simulink model "LQRconlacnguoc"  (R2024b)
settings: Solver=ode45  StartTime=0.0  StopTime=60  FixedStep=0.001  MaxStep=0.01  RelTol=1e-3
values from neighbouring files (symbols this model uses):
  D = [0; 0]    [K_vector_2.m]
libraries: simulink x20, slpidlib x11, slctrl_smc x5, mpclib x1, dspstat3 x1, rllib x1
(part 3 of 3)

== matlab function LQRconlacnguoc/Manual SMC Adaptive/Subsystem/MATLAB Function ==
  settings: updateMethod=DISCRETE  sampleTime=0.01
  data: s input; eta output; x input; x_ref input; phi output; C output
function [eta, phi, C] = culture_bees_smc(s, x, x_ref)

%% ── PREALLOCATE OUTPUTS ──────────────────────────────────────────────
eta = double(0);
phi = double(0);
C   = zeros(4, 1);

%% ── PERSISTENT STATE ─────────────────────────────────────────────────
persistent belief_lambda belief_alpha belief_mu
persistent norm_lambda norm_alpha norm_mu
persistent initialized

%% ── INITIALIZATION ───────────────────────────────────────────────────
if isempty(initialized)
    initialized   = int8(1);
    belief_lambda = double(8.0);
    belief_alpha  = double(20.0);
    belief_mu     = double(36.5);
    norm_lambda   = double([1.0,  15.0]);
    norm_alpha    = double([5.0,  25.0]);
    norm_mu       = double([10.0, 50.0]);
end

%% ── EXTRACT SCALARS ──────────────────────────────────────────────────
x2   = x(3);
xd2  = x(4);
x2r  = x_ref(3);
xd2r = x_ref(4);

e_pos = (x2r - x2)^2;
e_vel = (xd2r - xd2)^2;
e_tot = e_pos + e_vel;

%% ── DYNAMIC HARD FLOORS (key fix) ───────────────────────────────────
% Alpha floor scales directly with error magnitude
% When error is large, alpha CANNOT go below a meaningful minimum
% This replaces the soft adequacy penalty with a hard constraint
alpha_floor  = double(5.0) + double(15.0) * tanh(e_tot * 10.0);
% alpha_floor ≈ 5   when e_tot ≈ 0    (settled, allow alpha to relax)
% alpha_floor ≈ 20  when e_tot = 0.1  (moderate error, hold alpha high)
% alpha_floor ≈ 20  when e_tot large  (large error, maximum floor)

lambda_floor = double(1.0) + double(7.0)  * tanh(e_tot * 10.0);
% lambda_floor ≈ 1  when settled
% lambda_floor ≈ 8  when error present

% Enforce floors on belief state BEFORE optimization runs
% This prevents the optimizer from ever exploring below safe values
if belief_alpha < alpha_floor
    belief_alpha = alpha_floor;
end
if belief_lambda < lambda_floor
    belief_lambda = lambda_floor;
end

% Also enforce on normative bounds lower limit
current_alpha_min  = alpha_floor;
current_lambda_min = lambda_floor;

%% ── LOSS OF CONTROL RESET ────────────────────────────────────────────
control_lost = (e_tot > 0.005) && (belief_alpha < alpha_floor * 1.2);
if control_lost
    belief_lambda = double(8.0);
    belief_alpha  = double(20.0);
    belief_mu     = double(36.5);
    norm_lambda   = double([current_lambda_min, 15.0]);
    norm_alpha    = double([current_alpha_min,  25.0]);
    norm_mu       = double([10.0, 50.0]);
end

%% ── ALGORITHM HYPERPARAMETERS ────────────────────────────────────────
n_scout    = int32(10);
n_selected = int32(4);
n_recruit  = int32(20);
N_belief   = int32(5);

lambda_min = current_lambda_min;  lambda_max = double(15.0);
alpha_min  = current_alpha_min;   alpha_max  = double(25.0);
mu_min     = double(10.0);        mu_max     = double(50.0);

patch_alpha  = double(0.0125);
patch_lambda = double(0.0135);
patch_mu     = double(0.0175);

patch_c_alpha  = double(0.01);
patch_c_lambda = double(0.01);
patch_c_mu     = double(0.01);

%% ── PART 1: BREEDING ENGINE ──────────────────────────────────────────
scouts = zeros(n_scout, 3);
for i = 1:n_scout
    scouts(i,1) = norm_lambda(1) + rand()*(norm_lambda(2)-norm_lambda(1));
    scouts(i,2) = norm_alpha(1)  + rand()*(norm_alpha(2) -norm_alpha(1));
    scouts(i,3) = norm_mu(1)     + rand()*(norm_mu(2)    -norm_mu(1));
end

%% ── PART 2: SEARCH ENGINE ────────────────────────────────────────────
scout_mse = zeros(n_scout, 1);
for i = 1:n_scout
    scout_mse(i) = eval_mse(scouts(i,1), scouts(i,2), scouts(i,3), ...
                             s, x2, xd2, x2r, xd2r, e_tot, alpha_floor);
end

[~, idx]  = sort(scout_mse, 'ascend');
selected  = scouts(idx(1:n_selected), :);

best_recruit     = zeros(n_selected, 3);
best_recruit_mse = zeros(n_selected, 1);

for i = 1:n_selected
    site        = selected(i,:);
    recruits    = zeros(n_recruit, 3);
    recruit_mse = zeros(n_recruit, 1);

    for j = 1:n_recruit
        d_lambda = patch_lambda * site(1) * (rand() - 0.5);
        d_alpha  = patch_alpha  * site(2) * (rand() - 0.5);
        d_mu     = patch_mu     * site(3) * (rand() - 0.5);

        cl = clamp_val(site(1)+d_lambda, lambda_min, lambda_max);
        ca = clamp_val(site(2)+d_alpha,  alpha_min,  alpha_max);
        cm = clamp_val(site(3)+d_mu,     mu_min,     mu_max);

        recruits(j,:)  = [cl, ca, cm];
        recruit_mse(j) = eval_mse(cl, ca, cm, s, x2, xd2, x2r, xd2r, ...
                                   e_tot, alpha_floor);
    end

    [best_recruit_mse(i), best_j] = min(recruit_mse);
    best_recruit(i,:) = recruits(best_j,:);
end

[~, fittest_idx] = sort(best_recruit_mse, 'ascend');
fittest_bees     = best_recruit(fittest_idx, :);
fittest_mse_vec  = best_recruit_mse(fittest_idx);

%% ── PART 3: AGGREGATION KNOWLEDGE ENGINE ────────────────────────────
n_sc          = max(int32(1), round(0.4 * double(n_selected)));
scout_culture = fittest_bees(1:n_sc, :);
sc_mse        = fittest_mse_vec(1:n_sc);

n_scc       = max(int32(1), round(0.5 * double(n_sc)));
[~, sc_idx] = sort(sc_mse, 'ascend');
sel_culture = scout_culture(sc_idx(1:n_scc), :);

current_belief_mse = eval_mse(belief_lambda, belief_alpha, belief_mu, ...
                               s, x2, xd2, x2r, xd2r, e_tot, alpha_floor);
best_sc_mse = sc_mse(sc_idx(1));

if best_sc_mse < current_belief_mse
    belief_lambda = sel_culture(1,1);
    belief_alpha  = sel_culture(1,2);
    belief_mu     = sel_culture(1,3);
end

best_bl  = belief_lambda;
best_ba  = belief_alpha;
best_bm  = belief_mu;
best_mse = current_belief_mse;

for iter = 1:N_belief
    d_lc = patch_c_lambda * belief_lambda * (rand() - 0.5);
    d_ac = patch_c_alpha  * belief_alpha  * (rand() - 0.5);
    d_mc = patch_c_mu     * belief_mu     * (rand() - 0.5);

    cand_l = clamp_val(belief_lambda+d_lc, lambda_min, lambda_max);
    cand_a = clamp_val(belief_alpha +d_ac, alpha_min,  alpha_max);
    cand_m = clamp_val(belief_mu    +d_mc, mu_min,     mu_max);

    cand_mse = eval_mse(cand_l, cand_a, cand_m, s, x2, xd2, x2r, xd2r, ...
                         e_tot, alpha_floor);

    in_norm = (cand_l >= norm_lambda(1)) && (cand_l <= norm_lambda(2)) && ...
              (cand_a >= norm_alpha(1))  && (cand_a <= norm_alpha(2))  && ...
              (cand_m >= norm_mu(1))     && (cand_m <= norm_mu(2));

    if cand_mse < best_mse && in_norm
        best_bl  = cand_l;
        best_ba  = cand_a;
        best_bm  = cand_m;
        best_mse = cand_mse;
    end
end

% Update normative lower bounds to never go below current floors
norm_lambda = update_norm(norm_lambda, best_bl, lambda_min, lambda_max);
norm_alpha  = update_norm(norm_alpha,  best_ba, alpha_min,  alpha_max);
norm_mu     = update_norm(norm_mu,     best_bm, mu_min,     mu_max);

% Hard-enforce floors on updated bounds
if norm_lambda(1) < current_lambda_min
    norm_lambda(1) = current_lambda_min;
end
if norm_alpha(1) < current_alpha_min
    norm_alpha(1) = current_alpha_min;
end

belief_lambda = best_bl;
belief_alpha  = best_ba;
belief_mu     = best_bm;

%% ── FINAL FLOOR ENFORCEMENT ON OUTPUTS ──────────────────────────────
% Last line of defense — outputs never go below error-scaled floors
if belief_alpha  < alpha_floor;  belief_alpha  = alpha_floor;  end
if belief_lambda < lambda_floor; belief_lambda = lambda_floor; end

%% ── OUTPUT ASSIGNMENT ────────────────────────────────────────────────
eta = double(belief_alpha);
phi = double(1.0 / belief_mu);
C   = double(belief_lambda) .* [0.0; 1.0; 0.0; 1.0];

end

%% ════════════════════════════════════════════════════════════════════
%% LOCAL: MSE COST
%% ════════════════════════════════════════════════════════════════════
function mse = eval_mse(lambda, alpha, mu, s, x2, xd2, x2r, xd2r, ...
                         e_tot, alpha_floor)

    e_pos = (x2r - x2)^2;
    e_vel = (xd2r - xd2)^2;

    %% Term 1 — Tracking (primary)
    tracking = e_pos + e_vel;

    %% Term 2 — Surface penalty
    s_penalty = s^2;

    %% Term 3 — Alpha floor violation penalty
    % Heavily penalize any alpha below the error-scaled floor
    % This is what forces the optimizer to keep alpha adequate
    floor_violation = max(0.0, alpha_floor - alpha)^2 * 100.0;

    %% Term 4 — Chattering: only penalize when truly settled
    % settled = near surface AND near zero error simultaneously
    settled      = exp(-5.0 * abs(s)) * exp(-50.0 * e_tot);
    chat_penalty = alpha^2 * mu * settled * 0.0001;

    %% Term 5 — Lambda alignment with surface
    s_expected    = lambda * sqrt(e_pos + 0.0001) + sqrt(e_vel + 0.0001);
    align_penalty = (abs(s) - s_expected)^2 / (s_expected^2 + 0.01);

    %% Term 6 — Mu sizing (keep phi ≈ 0.0274, mu ≈ 36.5)
    % Penalize deviation from target mu
    mu_target   = double(36.5);
    mu_penalty  = (mu - mu_target)^2 / (mu_target^2) * 0.1;

    %% Weighted sum
    mse = 2.0  * tracking       ...
        + 0.3  * s_penalty      ...
        + 1.0  * floor_violation ...  % hardest constraint
        + 0.05 * chat_penalty   ...
        + 0.2  * align_penalty  ...
        + 0.1  * mu_penalty;

end

%% ════════════════════════════════════════════════════════════════════
%% LOCAL: CLAMP
%% ════════════════════════════════════════════════════════════════════
function val = clamp_val(val, lo, hi)
    if val < lo; val = lo; end
    if val > hi; val = hi; end
end

%% ════════════════════════════════════════════════════════════════════
%% LOCAL: NORMATIVE BOUNDS UPDATER
%% ════════════════════════════════════════════════════════════════════
function bounds = update_norm(bounds, best_val, hard_min, hard_max)
    shrink = double(0.005);        % very slow tightening
    range  = bounds(2) - bounds(1);
    new_lo = max(hard_min, bounds(1) + shrink*(best_val - bounds(1)));
    new_hi = min(hard_max, bounds(2) - shrink*(bounds(2) - best_val));
    if (new_hi - new_lo) < 0.4*range
        new_lo = max(hard_min, best_val - 0.2*range);
        new_hi = min(hard_max, best_val + 0.2*range);
    end
    bounds = [new_lo, new_hi];
end

== matlab function LQRconlacnguoc/Manual SMC Adaptive/Stable but chattery/MATLAB Function ==
  settings: updateMethod=DISCRETE  sampleTime=0.01
  data: s input; eta output; x input; x_ref input; phi output; C output
function [eta, phi, C] = culture_bees_smc(s, x, x_ref)

%% ── PREALLOCATE OUTPUTS ──────────────────────────────────────────────
eta = double(0);
phi = double(0);
C   = zeros(4, 1);

%% ── PERSISTENT STATE ─────────────────────────────────────────────────
persistent belief_lambda belief_alpha belief_mu
persistent norm_lambda norm_alpha norm_mu
persistent initialized

%% ── INITIALIZATION ───────────────────────────────────────────────────
if isempty(initialized)
    initialized   = int8(1);
    belief_lambda = double(8.0);
    belief_alpha  = double(20.0);
    belief_mu     = double(36.5);
    norm_lambda   = double([1.0,  15.0]);
    norm_alpha    = double([5.0,  25.0]);
    norm_mu       = double([10.0, 50.0]);
end

%% ── EXTRACT SCALARS ──────────────────────────────────────────────────
x2   = x(3);
xd2  = x(4);
x2r  = x_ref(3);
xd2r = x_ref(4);

e_pos = (x2r - x2)^2;
e_vel = (xd2r - xd2)^2;
e_tot = e_pos + e_vel;

%% ── DYNAMIC HARD FLOORS (key fix) ───────────────────────────────────
% Alpha floor scales directly with error magnitude
% When error is large, alpha CANNOT go below a meaningful minimum
% This replaces the soft adequacy penalty with a hard constraint
alpha_floor  = double(5.0) + double(15.0) * tanh(e_tot * 10.0);
% alpha_floor ≈ 5   when e_tot ≈ 0    (settled, allow alpha to relax)
% alpha_floor ≈ 20  when e_tot = 0.1  (moderate error, hold alpha high)
% alpha_floor ≈ 20  when e_tot large  (large error, maximum floor)

lambda_floor = double(1.0) + double(7.0)  * tanh(e_tot * 10.0);
% lambda_floor ≈ 1  when settled
% lambda_floor ≈ 8  when error present

% Enforce floors on belief state BEFORE optimization runs
% This prevents the optimizer from ever exploring below safe values
if belief_alpha < alpha_floor
    belief_alpha = alpha_floor;
end
if belief_lambda < lambda_floor
    belief_lambda = lambda_floor;
end

% Also enforce on normative bounds lower limit
current_alpha_min  = alpha_floor;
current_lambda_min = lambda_floor;

%% ── LOSS OF CONTROL RESET ────────────────────────────────────────────
control_lost = (e_tot > 0.005) && (belief_alpha < alpha_floor * 1.2);
if control_lost
    belief_lambda = double(8.0);
    belief_alpha  = double(20.0);
    belief_mu     = double(36.5);
    norm_lambda   = double([current_lambda_min, 15.0]);
    norm_alpha    = double([current_alpha_min,  25.0]);
    norm_mu       = double([10.0, 50.0]);
end

%% ── ALGORITHM HYPERPARAMETERS ────────────────────────────────────────
n_scout    = int32(10);
n_selected = int32(4);
n_recruit  = int32(20);
N_belief   = int32(5);

lambda_min = current_lambda_min;  lambda_max = double(15.0);
alpha_min  = current_alpha_min;   alpha_max  = double(25.0);
mu_min     = double(10.0);        mu_max     = double(50.0);

patch_alpha  = double(0.0125);
patch_lambda = double(0.0135);
patch_mu     = double(0.0175);

patch_c_alpha  = double(0.01);
patch_c_lambda = double(0.01);
patch_c_mu     = double(0.01);

%% ── PART 1: BREEDING ENGINE ──────────────────────────────────────────
scouts = zeros(n_scout, 3);
for i = 1:n_scout
    scouts(i,1) = norm_lambda(1) + rand()*(norm_lambda(2)-norm_lambda(1));
    scouts(i,2) = norm_alpha(1)  + rand()*(norm_alpha(2) -norm_alpha(1));
    scouts(i,3) = norm_mu(1)     + rand()*(norm_mu(2)    -norm_mu(1));
end

%% ── PART 2: SEARCH ENGINE ────────────────────────────────────────────
scout_mse = zeros(n_scout, 1);
for i = 1:n_scout
    scout_mse(i) = eval_mse(scouts(i,1), scouts(i,2), scouts(i,3), ...
                             s, x2, xd2, x2r, xd2r, e_tot, alpha_floor);
end

[~, idx]  = sort(scout_mse, 'ascend');
selected  = scouts(idx(1:n_selected), :);

best_recruit     = zeros(n_selected, 3);
best_recruit_mse = zeros(n_selected, 1);

for i = 1:n_selected
    site        = selected(i,:);
    recruits    = zeros(n_recruit, 3);
    recruit_mse = zeros(n_recruit, 1);

    for j = 1:n_recruit
        d_lambda = patch_lambda * site(1) * (rand() - 0.5);
        d_alpha  = patch_alpha  * site(2) * (rand() - 0.5);
        d_mu     = patch_mu     * site(3) * (rand() - 0.5);

        cl = clamp_val(site(1)+d_lambda, lambda_min, lambda_max);
        ca = clamp_val(site(2)+d_alpha,  alpha_min,  alpha_max);
        cm = clamp_val(site(3)+d_mu,     mu_min,     mu_max);

        recruits(j,:)  = [cl, ca, cm];
        recruit_mse(j) = eval_mse(cl, ca, cm, s, x2, xd2, x2r, xd2r, ...
                                   e_tot, alpha_floor);
    end

    [best_recruit_mse(i), best_j] = min(recruit_mse);
    best_recruit(i,:) = recruits(best_j,:);
end

[~, fittest_idx] = sort(best_recruit_mse, 'ascend');
fittest_bees     = best_recruit(fittest_idx, :);
fittest_mse_vec  = best_recruit_mse(fittest_idx);

%% ── PART 3: AGGREGATION KNOWLEDGE ENGINE ────────────────────────────
n_sc          = max(int32(1), round(0.4 * double(n_selected)));
scout_culture = fittest_bees(1:n_sc, :);
sc_mse        = fittest_mse_vec(1:n_sc);

n_scc       = max(int32(1), round(0.5 * double(n_sc)));
[~, sc_idx] = sort(sc_mse, 'ascend');
sel_culture = scout_culture(sc_idx(1:n_scc), :);

current_belief_mse = eval_mse(belief_lambda, belief_alpha, belief_mu, ...
                               s, x2, xd2, x2r, xd2r, e_tot, alpha_floor);
best_sc_mse = sc_mse(sc_idx(1));

if best_sc_mse < current_belief_mse
    belief_lambda = sel_culture(1,1);
    belief_alpha  = sel_culture(1,2);
    belief_mu     = sel_culture(1,3);
end

best_bl  = belief_lambda;
best_ba  = belief_alpha;
best_bm  = belief_mu;
best_mse = current_belief_mse;

for iter = 1:N_belief
    d_lc = patch_c_lambda * belief_lambda * (rand() - 0.5);
    d_ac = patch_c_alpha  * belief_alpha  * (rand() - 0.5);
    d_mc = patch_c_mu     * belief_mu     * (rand() - 0.5);

    cand_l = clamp_val(belief_lambda+d_lc, lambda_min, lambda_max);
    cand_a = clamp_val(belief_alpha +d_ac, alpha_min,  alpha_max);
    cand_m = clamp_val(belief_mu    +d_mc, mu_min,     mu_max);

    cand_mse = eval_mse(cand_l, cand_a, cand_m, s, x2, xd2, x2r, xd2r, ...
                         e_tot, alpha_floor);

    in_norm = (cand_l >= norm_lambda(1)) && (cand_l <= norm_lambda(2)) && ...
              (cand_a >= norm_alpha(1))  && (cand_a <= norm_alpha(2))  && ...
              (cand_m >= norm_mu(1))     && (cand_m <= norm_mu(2));

    if cand_mse < best_mse && in_norm
        best_bl  = cand_l;
        best_ba  = cand_a;
        best_bm  = cand_m;
        best_mse = cand_mse;
    end
end

% Update normative lower bounds to never go below current floors
norm_lambda = update_norm(norm_lambda, best_bl, lambda_min, lambda_max);
norm_alpha  = update_norm(norm_alpha,  best_ba, alpha_min,  alpha_max);
norm_mu     = update_norm(norm_mu,     best_bm, mu_min,     mu_max);

% Hard-enforce floors on updated bounds
if norm_lambda(1) < current_lambda_min
    norm_lambda(1) = current_lambda_min;
end
if norm_alpha(1) < current_alpha_min
    norm_alpha(1) = current_alpha_min;
end

belief_lambda = best_bl;
belief_alpha  = best_ba;
belief_mu     = best_bm;

%% ── FINAL FLOOR ENFORCEMENT ON OUTPUTS ──────────────────────────────
% Last line of defense — outputs never go below error-scaled floors
if belief_alpha  < alpha_floor;  belief_alpha  = alpha_floor;  end
if belief_lambda < lambda_floor; belief_lambda = lambda_floor; end

%% ── OUTPUT ASSIGNMENT ────────────────────────────────────────────────
eta = double(belief_alpha);
phi = double(1.0 / belief_mu);
C   = double(belief_lambda) .* [0.0; 1.0; 0.0; 1.0];

end

%% ════════════════════════════════════════════════════════════════════
%% LOCAL: MSE COST
%% ════════════════════════════════════════════════════════════════════
function mse = eval_mse(lambda, alpha, mu, s, x2, xd2, x2r, xd2r, ...
                         e_tot, alpha_floor)

    e_pos = (x2r - x2)^2;
    e_vel = (xd2r - xd2)^2;

    %% Term 1 — Tracking (primary)
    tracking = e_pos + e_vel;

    %% Term 2 — Surface penalty
    s_penalty = s^2;

    %% Term 3 — Alpha floor violation penalty
    % Heavily penalize any alpha below the error-scaled floor
    % This is what forces the optimizer to keep alpha adequate
    floor_violation = max(0.0, alpha_floor - alpha)^2 * 100.0;

    %% Term 4 — Chattering: only penalize when truly settled
    % settled = near surface AND near zero error simultaneously
    settled      = exp(-5.0 * abs(s)) * exp(-50.0 * e_tot);
    chat_penalty = alpha^2 * mu * settled * 0.0001;

    %% Term 5 — Lambda alignment with surface
    s_expected    = lambda * sqrt(e_pos + 0.0001) + sqrt(e_vel + 0.0001);
    align_penalty = (abs(s) - s_expected)^2 / (s_expected^2 + 0.01);

    %% Term 6 — Mu sizing (keep phi ≈ 0.0274, mu ≈ 36.5)
    % Penalize deviation from target mu
    mu_target   = double(36.5);
    mu_penalty  = (mu - mu_target)^2 / (mu_target^2) * 0.1;

    %% Weighted sum
    mse = 2.0  * tracking       ...
        + 0.3  * s_penalty      ...
        + 1.0  * floor_violation ...  % hardest constraint
        + 0.05 * chat_penalty   ...
        + 0.2  * align_penalty  ...
        + 0.1  * mu_penalty;

end

%% ════════════════════════════════════════════════════════════════════
%% LOCAL: CLAMP
%% ════════════════════════════════════════════════════════════════════
function val = clamp_val(val, lo, hi)
    if val < lo; val = lo; end
    if val > hi; val = hi; end
end

%% ════════════════════════════════════════════════════════════════════
%% LOCAL: NORMATIVE BOUNDS UPDATER
%% ════════════════════════════════════════════════════════════════════
function bounds = update_norm(bounds, best_val, hard_min, hard_max)
    shrink = double(0.005);        % very slow tightening
    range  = bounds(2) - bounds(1);
    new_lo = max(hard_min, bounds(1) + shrink*(best_val - bounds(1)));
    new_hi = min(hard_max, bounds(2) - shrink*(bounds(2) - best_val));
    if (new_hi - new_lo) < 0.4*range
        new_lo = max(hard_min, best_val - 0.2*range);
        new_hi = min(hard_max, best_val + 0.2*range);
    end
    bounds = [new_lo, new_hi];
end

== matlab function LQRconlacnguoc/Subsystem/MATLAB Function2 ==
  settings: updateMethod=DISCRETE
  data: x1 input; Ki_out output; x2 input; v1 input; v2 input; x2_ref input
function Ki_out = adaptive_Ki(x1, x2, v1, v2, x2_ref)
    persistent Ki_current e_int;
    
    % Your requested baseline and limits
    baseline_Ki = 900; 
    max_Ki = 1200; 
    min_Ki = 900; 
    
    % 1. INITIALIZATION 
    if isempty(Ki_current)
        Ki_current = baseline_Ki; 
        e_int = [0; 0; 0; 0]; 
    end
    
    % 2. DEFINE TARGETS
    ref_x1 = 0; 
    ref_x2 = x2_ref; 
    ref_v1 = 0; 
    ref_v2 = 0;
    
    % 3. CALCULATE CURRENT ERROR
    e = [(ref_x1 - x1); (ref_x2 - x2); (ref_v1 - v1); (ref_v2 - v2)];
    dt = 0.01; 
    
    % 4. CONDITIONAL INTEGRATION (THE FIX)
    % Only accumulate error if the car is within 5cm of the target.
    % If it's making a big jump (like 0.4 to 0.1), flush the memory to 0.
    if abs(e(2)) < 0.05
        e_int = e_int + (e * dt);
    else
        e_int = [0; 0; 0; 0];
    end
    
    % Tighter Anti-Windup clamp (100 was way too high for a 0.4m system)
    e_int = max(min(e_int, 1), -1); 
    
    % 5. CALCULATE THE ADAPTIVE METRIC
    integral_metric = abs(e' * e_int); 
    
    % 6. YOUR REQUESTED PARAMETERS
    alpha_2 = 50;  % 0.5e2
    sigma = 5;     % Heavy leakage
    
    % 7. THE GRADIENT UPDATE RULE WITH LEAKAGE
    delta_Ki = (alpha_2 * integral_metric) - (sigma * (Ki_current - baseline_Ki));
    
    Ki_current = Ki_current + (delta_Ki * dt);
    
    % 8. SAFETY CLAMP 
    if Ki_current > max_Ki
        Ki_current = max_Ki;
    elseif Ki_current < min_Ki
        Ki_current = min_Ki;
    end
    
    Ki_out = Ki_current;
end

== matlab function LQRconlacnguoc/Reward ==
  data: x2 input; x2_ref input; u input; reward output; time_since_change input; x2_prev input; next_x2_prev output
function [reward, next_x2_prev] = calc_reward(x2, x2_ref, u, time_since_change, x2_prev)
    
    % Initialize base reward (survival bonus)
    reward = 0.1; 
    x2_error = abs(x2_ref - x2);
    delta_x2 = abs(x2 - x2_prev);
    
    % --- 1. TIGHT BOUNDARY BLEED (0.0020m) ---
    % Standard proportional penalty for error
    reward = reward - (10 * x2_error^2); 
    
    % The "Bleed": Harsh flat penalty every 0.01s it is outside the tight boundary
    if x2_error > 0.0020
        reward = reward - 1.0; 
    else
        % Give it a nice dopamine hit for staying perfectly on target
        reward = reward + 2.0; 
    end
    
    % --- 2. SMC ROBUSTNESS (Settle-Time Grace Period) ---
    % Only enforce strict vibration limits AFTER 1.0 second of a new reference jump
    if time_since_change > 1.0
        % If it moves more than 5mm in a single 0.01s step (violent shaking)
        if delta_x2 > 0.005
            % Massive penalty to teach it to hold still like an SMC
            reward = reward - 5.0; 
        end
    end
    
    % --- 3. ENERGY EFFICIENCY ---
    % Normalize u to your 3500N max, then square it.
    % This forces the AI to use the absolute minimum force required.
    reward = reward - 0.5 * ((u / 3500)^2);
    
    % Pass the current x2 to the next step
    next_x2_prev = x2; 

    % Calculate how much the AI tried to change the force
    delta_u = abs(u - u_prev);
    
    % --- 4. HARDWARE LIMIT PENALTY (250N/step) ---
    if delta_u > 250
        % If it asks for 300N, it is 50N over the limit. 
        % We square the violation so massive jumps cause massive pain.
        violation = delta_u - 250;
        reward = reward - (violation^2); 
    end
end

== matlab function LQRconlacnguoc/IsDone ==
  data: x1 input; is_done output; x2 input; x2_ref input; next_timer_03 output; timer_03 input; time_since_change input; current_step_size input; x2_ref_prev input; next_time_since_change output; next_step_size output; next_ref_prev output
function [is_done, next_timer_03, next_time_since_change, next_step_size, next_ref_prev] = check_safety(x1, x2, x2_ref, timer_03, time_since_change, current_step_size, x2_ref_prev)
    
    dt = 0.01; 
    is_done = false;
    x2_error = x2_ref - x2;
    
    % --- 1. DETECT A REFERENCE CHANGE ---
    % If the reference changes by more than 1mm, reset our dynamic timers
    if abs(x2_ref - x2_ref_prev) > 0.001
        next_time_since_change = 0;
        next_step_size = abs(x2_ref - x2_ref_prev); % Store how big the jump was
    else
        next_time_since_change = time_since_change + dt;
        next_step_size = current_step_size; % Keep remembering the jump size
    end
    next_ref_prev = x2_ref; % Pass current ref to next step
    
    % --- 2. INSTANT DEATH CONDITIONS ---
    if abs(x1) > 0.65
        is_done = true;
        next_timer_03 = 0; return;
    end
    
    % --- 3. ANTI-CHEAT: 0.3m error for 0.75s ---
    if abs(x2_error) > 0.3
        next_timer_03 = timer_03 + dt;
    else
        next_timer_03 = 0; % Reset instantly if it dips back into the safe zone
    end
    
    if next_timer_03 > 0.75
        is_done = true; 
    end
    
    % --- 4. DYNAMIC RISE TIME LIMIT ---
    % Allowed time = step_size * 2.2 seconds. (e.g., 0.3m jump = 0.66s allowed)
    % If there hasn't been a jump yet, default to a reasonable limit (e.g., 2 seconds)
    if next_step_size > 0
        allowed_settle_time = next_step_size * 2.2;
    else
        allowed_settle_time = 2.0; 
    end
    
    % If time is up, it MUST be within the 0.020m boundary
    if (next_time_since_change > allowed_settle_time) && (abs(x2_error) > 0.020)
        is_done = true;
    end
end
